simulink model "stm32_delay_optimization_stage2_working"  (R2025a)
settings: Solver=FixedStepDiscrete  StartTime=0.0  StopTime=inf  FixedStep=0.01  RelTol=1e-3  EnableMultiTasking=on
libraries: canmsglib x4, stm32blockslib x2, simulink x1, stm32f1xxblockslib x1
settings Model: STM32="{\"DigitalPortWrite\":[{\"ID\":\"LED:2\"},{\"ID\":\"LED:3\"}],\"CANWrite\":[{\"ID\":\"LED:5\"},{\"ID\":\"ESP_Controller_STM32:5\"},{\"ID\":\"ESP_Controller_STM32_test1:5\"},{\"ID\":\"ESP_Controller_STM32_test1_error_validation:36\"},{\"ID\":\"ESP_Controller_STM32_test1_seq_sync:36\"},{\"ID\":\"version2_codex_ESP_Controller_STM32_test1_seq_sync_buildable:36\"},{\"ID\":\"STM32_seq_sync_portable:36\"},{\"ID\":\"stm32backup111:36\"},{\"ID\":\"stm32_delay_optimization_stage2_working:36\"}],\"CANRead\":[{\"ID\":\"LED:7\"},{\"ID\":\"ESP_Controller_STM32:7\"},{\"ID\":\"ESP_Controller_STM32_test1:7\"},{\"ID\":\"ESP_Controller_STM32_test1_error_validation:7\"},{\"ID\":\"ESP_Controller_STM32_test1_seq_sync:7\"},{\"ID\":\"version2_codex_ESP_Controller_STM32_test1_seq_sync_buildable:7\"},{\"ID\":\"STM32_seq_sync_portable:7\"},{\"ID\":\"stm32backup111:7\"},{\"ID\":\"stm32_delay_optimization_stage2_working:7\"}],\"HardwareInterrupt\":[{\"ID\":\"ESP_Controller_STM32_test1:28\"},{\"ID\":\"STM32_seq_sync_portable:28\"},{\"ID\":\"stm32backup111:28\"}]}"  Creator=65365  LastModifiedBy=65365
settings OptimizationCC: DefaultParameterBehavior=Inlined  EnhancedBackFolding=on  PassReuseOutputArgsAs=Individual arguments  ZeroExternalMemoryAtStartup=off  ZeroInternalMemoryAtStartup=off  MaxStackSize=512  OptimizeBlockOrder=speed  DifferentSizesBufferReuse=on  OptimizationCustomize=off  EfficientTunableParamExpr=on
settings DebuggingCC: ParameterTunabilityLossMsg=error
settings HardwareCC: ProdBitPerPointer=32.0  ProdBitPerSizeT=32.0  ProdBitPerPtrDiffT=32.0  ProdLargestAtomicInteger=Long  ProdLargestAtomicFloat=Double  ProdWordSize=32.0  ProdLongLongMode=on  ProdHWDeviceType=ARM Compatible->ARM Cortex-M
settings SFSimCC: MATLABDynamicMemAlloc=off
settings RTWCC: SystemTargetFile=ert.tlc  HardwareBoard=STM32F1xx Based  TemplateMakefile=ert_default_tmf  PostCodeGenCommand=codertarget.postCodeGenHookCommand(h); addpath('D:\\Lab\\step1'); fix_stm32_can_fifo_release_hook();  Toolchain=GNU Tools for ARM Embedded Processors  Description=Embedded Coder
settings CodeAppCC: ForceParamTrailComments=on  IgnoreCustomStorageClasses=off  OperatorAnnotations=on  SimulinkDataObjDesc=on  SFDataObjDesc=on  InsertBlockDesc=on
settings ERTTargetCC: ExtModeTransport=3.0  ExtModeStaticAllocSize=2048.0  TargetLangStandard=C99 (ISO)  CodeReplacementLibrary=ARM Cortex-M

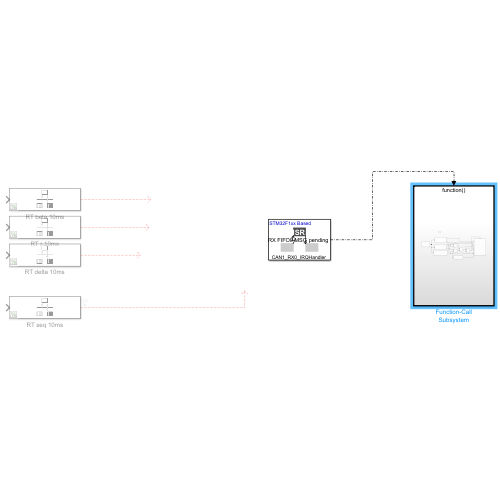
[thumbnail: Simulink's stored preview of the top-level diagram]
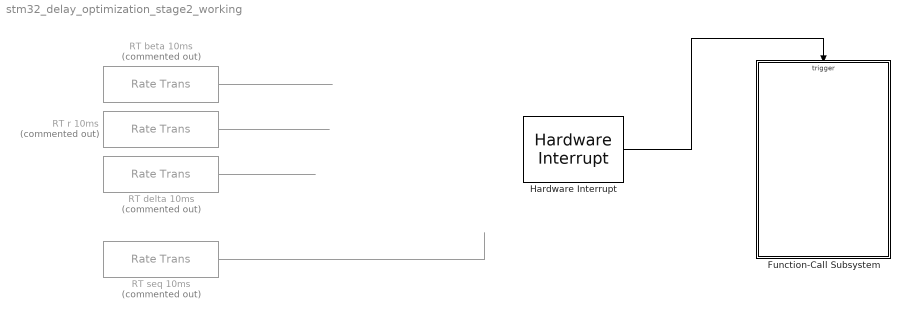
== system stm32_delay_optimization_stage2_working ==
  Function-Call Subsystem : Subsystem  TreatAsAtomicUnit=on
  Hardware Interrupt : stm32f1xxblockslib/Hardware Interrupt  ISRGroup=Controller Area Network (CAN)  ISRName=CAN1_RX0_IRQHandler  ISRNumber=35  EventsList={ 'off', 'CAN1 RX FIFO0 OVR', '1'; 'off', 'CAN1 RX FIFO0 Full', '2'; 'on', 'CAN1 RX FIFO0 MSG pending', '3'; 'off', 'Custom event', '4' }  SelectedEvents={'CAN1 RX FIFO0 MSG pending'}  TaskPriority=30  DisablePreemption=off  ClearInterruptFlagsAtEndOfEvent=on  InterruptDefinitionFile=$(TARGET_ROOT)/registry/interrupts/STM32F1xxBased_interrupts.xml  HardwareBoard=STM32F1xx Based  EnableSimPort=off
  RT beta 10ms : RateTransition  Commented=on  Deterministic=off  OutPortSampleTime=0.01
  RT delta 10ms : RateTransition  Commented=on  Deterministic=off  OutPortSampleTime=0.01
  RT r 10ms : RateTransition  Commented=on  Deterministic=off  OutPortSampleTime=0.01
  RT seq 10ms : RateTransition  Commented=on  Deterministic=off  OutPortSampleTime=0.01
  wires:
  Hardware Interrupt/1 -> Function-Call Subsystem/Trigger
  RT beta 10ms/1 -> ?
  RT delta 10ms/1 -> ?
  RT seq 10ms/1 -> ?
  RT r 10ms/1 -> ?

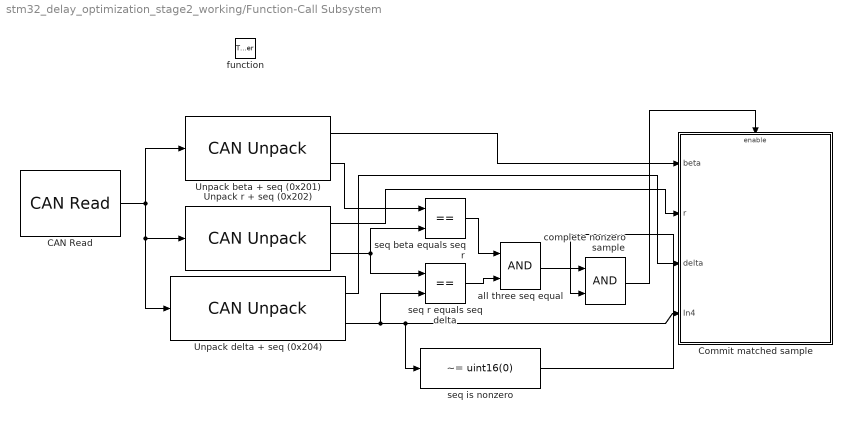
== system stm32_delay_optimization_stage2_working/Function-Call Subsystem ==
  function : TriggerPort  TriggerType=function-call  VariantControl=(inherit)
  CAN Read : stm32blockslib/CAN Read  CANModule=CAN1  BlockMode=Receive  OperationReadMode=Data  OperationWriteMode=Data  OutputTypeReadMode=Packed  DataFormatWriteMode=Raw data  ReadSource=FIFO 0  IdentifierTypeVia=Dialog  IdentifierType=Standard (11-bit identifier)  IdentifierVia=Inport  Identifier=100  DataLengthVia=Inport  DataLength=8  OutputIdType=off  TransmitRemoteFrame=off  OutputRemoteFrame=off  OutputTxFifoLevel=off  OutputRxFifoLevel=off  OutputStatus=off  Timeout=0  SampleTime=-1
      settings: LibrarySourceBlock=stm32f1xxblockslib/CAN Read
  Commit matched sample : Subsystem
  Unpack beta + seq (0x201) : canmsglib/CAN Unpack  CANdbFile=D:\Lab\step1\vehicle_controller.dbc  MsgList=Controller_Input  MsgName=Controller_Input  MsgIDType=Standard (11-bit identifier)  MsgIdentifier=513  MsgLength=6  SignalInfo="{ 'beta', '0', '32', 'LE', 'single', 'Standard', '0', '1', '0', '-Inf', 'Inf';     'seq_beta', '32', '16', 'LE', 'unsigned', 'Standard', '0', '1', '0', '0', '65535' }"  IDPort=off  TimestampPort=off  ErrorPort=off  RemotePort=off  LengthPort=off  StatusPort=off  ApplyMinMax=off
      settings: LibrarySourceBlock=canlib/CAN Unpack
  Unpack delta + seq (0x204) : canmsglib/CAN Unpack  CANdbFile=D:\Lab\step1\vehicle_controller.dbc  MsgList=Controller_Input  MsgName=Controller_Input  MsgIDType=Standard (11-bit identifier)  MsgIdentifier=516  MsgLength=6  SignalInfo="{ 'delta', '0', '32', 'LE', 'single', 'Standard', '0', '1', '0', '-Inf', 'Inf';     'seq_delta', '32', '16', 'LE', 'unsigned', 'Standard', '0', '1', '0', '0', '65535' }"  IDPort=off  TimestampPort=off  ErrorPort=off  RemotePort=off  LengthPort=off  StatusPort=off  ApplyMinMax=off
      settings: LibrarySourceBlock=canlib/CAN Unpack
  Unpack r + seq (0x202) : canmsglib/CAN Unpack  CANdbFile=D:\Lab\step1\vehicle_controller.dbc  MsgList=Controller_Input  MsgName=Controller_Input  MsgIDType=Standard (11-bit identifier)  MsgIdentifier=514  MsgLength=6  SignalInfo={ 'yaw_rate', '0', '32', 'LE', 'single', 'Standard', '0', '1', '0', '-Inf', 'Inf'; 'seq_r', '32', '16', 'LE', 'unsigned', 'Standard', '0', '1', '0', '0', '65535' }  IDPort=off  TimestampPort=off  ErrorPort=off  RemotePort=off  LengthPort=off  StatusPort=off  ApplyMinMax=off
      settings: LibrarySourceBlock=canlib/CAN Unpack
  all three seq equal : Logic  AllPortsSameDT=off  OutDataTypeStr=boolean
  complete nonzero sample : Logic  AllPortsSameDT=off  OutDataTypeStr=boolean
  seq beta equals seq r : RelationalOperator  Operator===  OutDataTypeStr=boolean  RndMeth=Simplest  InputSameDT=off
  seq is nonzero : simulink/Logic and Bit Operations/Compare To Constant  relop=~=  const=uint16(0)  OutDataTypeStr=boolean
  seq r equals seq delta : RelationalOperator  Operator===  OutDataTypeStr=boolean  RndMeth=Simplest  InputSameDT=off
  wires:
  CAN Read/1 -> Unpack r + seq (0x202)/1, Unpack delta + seq (0x204)/1, Unpack beta + seq (0x201)/1
  Unpack beta + seq (0x201)/2 -> seq beta equals seq r/1
  Unpack r + seq (0x202)/2 -> seq beta equals seq r/2, seq r equals seq delta/1
  Unpack delta + seq (0x204)/2 -> seq r equals seq delta/2, Commit matched sample/4(In4), seq is nonzero/1
  seq beta equals seq r/1 -> all three seq equal/1
  seq r equals seq delta/1 -> all three seq equal/2
  all three seq equal/1 -> complete nonzero sample/1
  Unpack beta + seq (0x201)/1 -> Commit matched sample/1(beta)
  Unpack r + seq (0x202)/1 -> Commit matched sample/2(r)
  Unpack delta + seq (0x204)/1 -> Commit matched sample/3(delta)
  seq is nonzero/1 -> complete nonzero sample/2
  complete nonzero sample/1 -> Commit matched sample/Enable

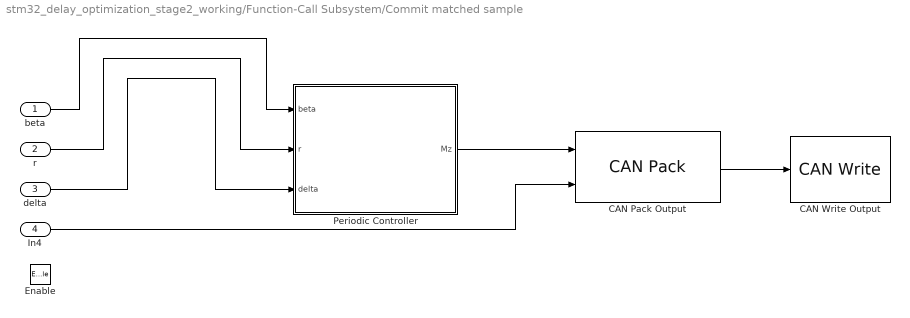
== system stm32_delay_optimization_stage2_working/Function-Call Subsystem/Commit matched sample ==
  beta : Inport
  r : Inport  Port=2
  delta : Inport  Port=3
  In4 : Inport  Port=4
  Enable : EnablePort
  CAN Pack Output : canmsglib/CAN Pack  Priority=5  CANdbFile=D:\Lab\step1\vehicle_controller.dbc  MsgList=Controller_Output  MsgName=Controller_Output  MsgIDType=Standard (11-bit identifier)  MsgIdentifier=515  CANIDInput=off  MsgLength=6  Remote=off  ApplyMinMax=off  BusOutput=on  SignalInfo="{ 'M', '0', '32', 'LE', 'single', 'Standard', '0', '1', '0', '-Inf', 'Inf';          'sample_seq', '32', '16', 'LE', 'unsigned', 'Standard', '0', '1', '0', '0', '65535' }"
      settings: LibrarySourceBlock=canlib/CAN Pack  DataFormat=manually specified signals
  CAN Write Output : stm32blockslib/CAN Write  Priority=6  CANModule=CAN1  BlockMode=Transmit  OperationReadMode=Data  OperationWriteMode=Data  OutputTypeReadMode=Unpacked  DataFormatWriteMode=CAN Message  ReadSource=FIFO 0  IdentifierTypeVia=Dialog  IdentifierType=Standard (11-bit identifier)  IdentifierVia=Dialog  Identifier=hex2dec('203')  DataLengthVia=Dialog  DataLength=6  OutputIdType=off  TransmitRemoteFrame=off  OutputRemoteFrame=off  OutputTxFifoLevel=off  OutputRxFifoLevel=off  OutputStatus=off  Timeout=0.001  SampleTime=-1
      settings: LibrarySourceBlock=stm32f1xxblockslib/CAN Write
  Periodic Controller : MATLAB Function  Priority=4  TreatAsAtomicUnit=on
  wires:
  beta/1 -> Periodic Controller/1(beta)
  r/1 -> Periodic Controller/2(r)
  delta/1 -> Periodic Controller/3(delta)
  In4/1 -> CAN Pack Output/2
  Periodic Controller/1(Mz) -> CAN Pack Output/1
  CAN Pack Output/1 -> CAN Write Output/1

== matlab function stm32_delay_optimization_stage2_working/Function-Call Subsystem/Commit matched sample/Periodic Controller ==
  data: beta input; r input; delta input; Mz output
function Mz = direct_lyapunov_controller(beta, r, delta)
    % 1. 车辆参数定义 
    m = 1750; Iz = 3000; a = 1.25; b = 1.45;
    kf = 65000; kr = 45000; vx = 30;
    
    % 2. 设定期望的能量耗散速度 (可调参数)
    K1 = 500000;         % 对应 beta 的衰减力度
    K2 = 500000;         % 对应 r 的衰减力度
    epsilon = 0.00001;    % 极小保护阈值
    % 3. 实时计算当前轮胎侧向力
    Fyf = kf * (delta - beta - a * r / vx);
    Fyr = kr * (-beta + b * r / vx);

    if abs(r) < epsilon
        if r >= 0
            r_safe = epsilon;
        else
            r_safe = -epsilon;
        end
    else
        r_safe = r;
    end
    
    % 4. 严格执行李雅普诺夫代数解公式
    term1 = -K1 * beta^2 - K2 * r_safe^2;
    term2 = -2 * beta * (Fyf + Fyr - m * vx * r_safe);
    
    Mz_raw = (term1 + term2) /(2 * r_safe )  - (a * Fyf - b * Fyr);
    
    % 5. 物理限幅 
    if Mz_raw > 4000
        Mz = 4000;
    elseif Mz_raw < -4000
        Mz = -4000;
    else
        Mz = Mz_raw;
    end
end
